simulink model "reduce_emf_user_cleanup"  (R2024b)
settings: Solver=FixedStepAuto  StartTime=0.0  StopTime=10  FixedStep=Tsim  RelTol=1e-4  EnableMultiTasking=on
InitFcn:
  | clc;
  | clear;
  | %% Parameters of the motor
  | Tsim = 1e-6;
  | Tpwm=1e-4;
  | Ts = 1e-4;
  | R = 1.8665;
  | Rs=1.8665;
  | Ls=8.96e-3;
  | Ld = 8.96e-3;
  | Lq = 8.96e-3;
  | L1=(Ld +Lq )/2;
  | L2=(Lq -Ld )/2;
  | flux = 0.21;
  | F=0.00008;
  | J=0.003;
  | Np=4;
  | fpwm = 10e3;
  | Vdc=311;
  | wn=100;
  | %% Controller limiter                                                           % Maximum torque (Nm)
  | I_max = 7.5;                                                    % Maximum current (A)
  | V_max = Vdc/sqrt(3);
  | 
  | 
  | %% 转速环电流环带宽
  | wspd=20;
  | wcur=500;
  | 
  | %% LESO
  | w0=10000;
  | beta1=2*w0-R/Ld;
  | beta2=w0*w0;
  | %% IF启动
  | Iq_if=7;
  | we_if_acc=300;
  | we_if_max=180;
  | we_switch=150;
model workspace (MAT data in the model file):
  new = 0
undefined symbols (not defined in the file or in its folder): DiscIntNeverNeededParam, dspblkCoreblockFVToolHelper, gcbh
libraries: spsDCVoltageSourceLib x1, spsGroundLib x1, spsPermanentMagnetSynchronousMachineLib x1, spsUniversalBridgeLib x1, spspowerguiLib x1, simulink x1
(part 1 of 2)
settings Model: SimulationMode=accelerator  Creator=Lenovo  LastModifiedBy=azx
settings SolverCC: AlgebraicLoopSolver=TrustRegion
settings DataIOCC: ReturnWorkspaceOutputs=off
settings OptimizationCC: ReuseModelBlockBuffer=off
settings DebuggingCC: UnconnectedInputMsg=warning  UnconnectedOutputMsg=warning  UnconnectedLineMsg=warning
settings ModelReferenceCC: EnableRefExpFcnMdlSchedulingChecks=on
settings RTWCC: GPUComputeCapability=3.5

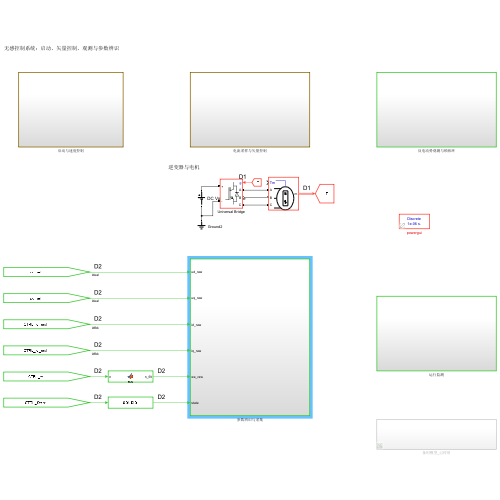
[thumbnail: Simulink's stored preview of the top-level diagram]
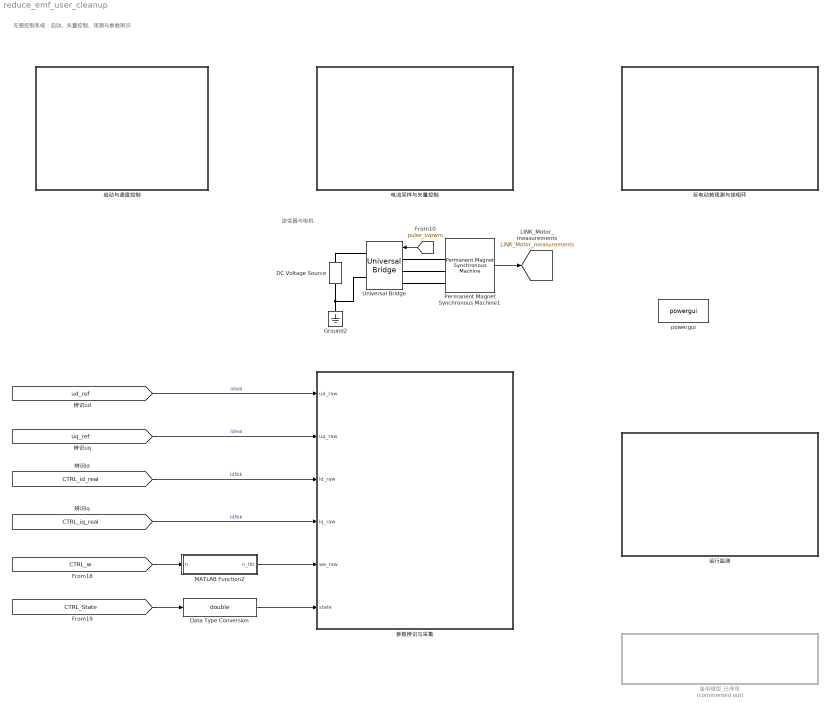
== system reduce_emf_user_cleanup ==
  note: 无感控制系统：启动、矢量控制、观测与参数辨识
  note: 逆变器与电机
  DC Voltage Source : spsDCVoltageSourceLib/DC Voltage Source  Amplitude=Vdc  Measurements=None
  Data Type Conversion : DataTypeConversion  OutDataTypeStr=double  SaturateOnIntegerOverflow=off  RndMeth=Floor
  Ground2 : spsGroundLib/Ground  LConnTagsString=a
  MATLAB Function2 : MATLAB Function  TreatAsAtomicUnit=on
  Permanent Magnet Synchronous Machine1 : spsPermanentMagnetSynchronousMachineLib/Permanent Magnet Synchronous Machine  NbPhases=3  FluxDistribution=Sinusoidal  RotorType=Salient-pole  MechanicalLoad=Torque Tm  PresetModel=No  ShowDetailedParameters=on  MeasurementBus=off  Resistance=R  Inductance=8.5e-3  dqInductances=[Ld,Lq]  La=Ld  MachineConstant=Flux linkage established by magnets (V.s)  Flux=0.21  VoltageCst=152.3591  TorqueCst=1.26  Flat=120  Mechanical=[0.03 2e-2 Np 0]  PolePairs=4  InitialConditions=[0,0, 0,0]  InitialConditions5ph=[0 0 0 0 0 0]  RefAngle=Aligned with phase A axis (original Park)  IterativeDiscreteModel=Trapezoidal non iterative  TsBlock=-1  TsPowergui=0
  Universal Bridge : spsUniversalBridgeLib/Universal Bridge  Arms=3  SnubberResistance=1e5  SnubberCapacitance=inf  Device=IGBT / Diodes  Ron=1e-3  Lon=0  ForwardVoltages="[  0  0  ]"  ForwardVoltage=0  GTOparameters=[ 10e-6 , 20e-6 ]  IGBTparameters=[ 1e-6 , 2e-6 ]  Measurements=None  Measurements_2=None  converterType=Rectifier
  powergui : spspowerguiLib/powergui  Priority=1  SimulationMode=Discrete  SampleTime=Tsim  frequency=60  Iterations=50  frequencyindice=0  Pbase=100e6  ErrMax=1e-4  UnitsV=kV  UnitsW=MW  buscounter=0  FunctionMessages=off  echomessages=off  EnableUseOfTLC=off  CurrentSourceSwitches=off  DisableSnubberDevices=off  DisableRonSwitches=off  DisableVfSwitches=off  DisplayEquations=off  AutomaticDiscreteSolvers=off  SolverType=Tustin/Backward Euler (TBE)  Interpol=off  ExternalGateDelay=off  methode=off  Ts=100  x0status=blocks  SPID=on  SwTol=0  HookPort=off  NonlinearTolerance=1e-4  nMaxIteration=100  ContinueOnMaxIteration=off  RestoreLinks=warning  ResistiveCurrentMeasurement=off  Frange=[0:2:500]  Ylog=off  Xlog=on  ShowGrid=off  save=off  variable=ZData  structure=0  ZoomFFT=off  StartTime=0.0  cycles=1  DisplayStyle=1  fundamental=60  FreqAxis=off  MaxFrequency=1000  frequencyindicesteady=1  RmsSteady=1  display=off
  参数辨识与采集 : Subsystem
  反电动势观测与锁相环 : Subsystem  Description=仅整理原计算块与信号标签；虚拟子系统，不增加采样、延迟或执行条件。
  启动与速度控制 : Subsystem  Description=仅整理原计算块与信号标签；虚拟子系统，不增加采样、延迟或执行条件。
  备用模型_已停用 : Subsystem  Commented=on
  电流采样与矢量控制 : Subsystem  Description=仅整理原计算块与信号标签；虚拟子系统，不增加采样、延迟或执行条件。
  运行监测 : Subsystem  Description=仅整理原计算块与信号标签；虚拟子系统，不增加采样、延迟或执行条件。
  tag scope: LINK_Motor_measurements=global
  wires:
  [pulse_svpwm] -> Universal Bridge/1
  Permanent Magnet Synchronous Machine1/1 -> [LINK_Motor_measurements]
  [CTRL_w] -> MATLAB Function2/1(n)
  [CTRL_State] -> Data Type Conversion/1
  [ud_ref] -> 参数辨识与采集/1(ud_raw)  "ideal"
  [uq_ref] -> 参数辨识与采集/2(uq_raw)  "ideal"
  [CTRL_id_real] -> 参数辨识与采集/3(id_raw)  "idfbk"
  [CTRL_iq_real] -> 参数辨识与采集/4(iq_raw)  "idfbk"
  MATLAB Function2/1(n_filt) -> 参数辨识与采集/5(we_raw)
  Data Type Conversion/1 -> 参数辨识与采集/6(state)
  connections:
  DC Voltage Source/RConn1 -- Universal Bridge/RConn1
  Permanent Magnet Synchronous Machine1/LConn1 -- Universal Bridge/LConn1
  Permanent Magnet Synchronous Machine1/LConn2 -- Universal Bridge/LConn2
  Permanent Magnet Synchronous Machine1/LConn3 -- Universal Bridge/LConn3
  Universal Bridge/RConn2 -- DC Voltage Source/LConn1 -- Ground2/LConn1

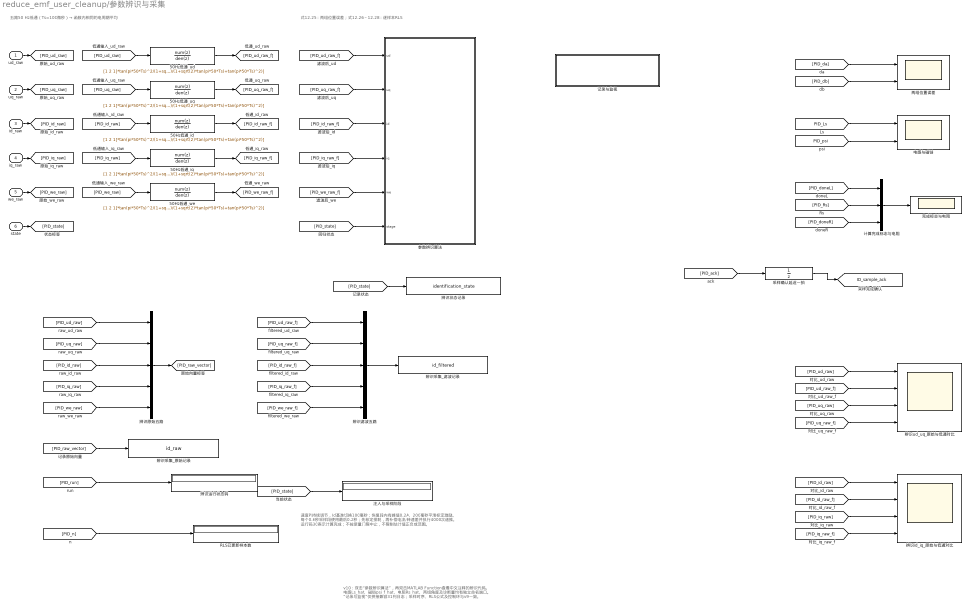
== system reduce_emf_user_cleanup/参数辨识与采集 ==
  note: 五路50 Hz低通（Ts=100微秒）→ 函数内相同的电周期平均
  note: 式12.25：两组位置误差；式12.26～12.28：逐样本RLS
  note: 速度PI持续调节，Id基准切换100毫秒；恢复段内有峰值0.2A、200毫秒平滑标定激励。
      | 每个0.6秒采样段使用最后0.2秒；先标定损耗，再补偿电流/转速差并执行4000次递推。
      | 运行码30表示计算完成；不按质量门限中止，不限制估计值正负或范围。
  note: v10：双击“参数辨识算法”，再双击MATLAB Function查看中文注释的辨识代码。
      | 电感Ls_hat、磁链psi_f_hat、电阻Rs_hat、两组角度及诊断量均有独立命名端口。
      | “记录与监视”仅拼接兼容31列日志；采样时序、RLS公式及控制环与v9一致。
  ud_raw : Inport
  uq_raw : Inport  Port=2
  id_raw : Inport  Port=3
  iq_raw : Inport  Port=4
  we_raw : Inport  Port=5
  state : Inport  Port=6
  50Hz低通_id : DiscreteTransferFcn  Description=输入已是Ts=100us；同速率二阶Butterworth低通，不作升采样，不声称恢复上游已混叠信息。  Numerator=[1 2 1]*tan(pi*50*Ts)^2/(1+sqrt(2)*tan(pi*50*Ts)+tan(pi*50*Ts)^2)  Denominator=[1 2*(tan(pi*50*Ts)^2-1)/(1+sqrt(2)*tan(pi*50*Ts)+tan(pi*50*Ts)^2) (1-sqrt(2)*tan(pi*50*Ts)+tan(pi*50*Ts)^2)/(1+sqrt(2)*tan(pi*50*Ts)+tan(pi*50*Ts)^2)]  SampleTime=Ts
  50Hz低通_iq : DiscreteTransferFcn  Description=输入已是Ts=100us；同速率二阶Butterworth低通，不作升采样，不声称恢复上游已混叠信息。  Numerator=[1 2 1]*tan(pi*50*Ts)^2/(1+sqrt(2)*tan(pi*50*Ts)+tan(pi*50*Ts)^2)  Denominator=[1 2*(tan(pi*50*Ts)^2-1)/(1+sqrt(2)*tan(pi*50*Ts)+tan(pi*50*Ts)^2) (1-sqrt(2)*tan(pi*50*Ts)+tan(pi*50*Ts)^2)/(1+sqrt(2)*tan(pi*50*Ts)+tan(pi*50*Ts)^2)]  SampleTime=Ts
  50Hz低通_ud : DiscreteTransferFcn  Description=输入已是Ts=100us；同速率二阶Butterworth低通，不作升采样，不声称恢复上游已混叠信息。  LoadFcn=dspblkCoreblockFVToolHelper(gcbh,'load');  Numerator=[1 2 1]*tan(pi*50*Ts)^2/(1+sqrt(2)*tan(pi*50*Ts)+tan(pi*50*Ts)^2)  Denominator=[1 2*(tan(pi*50*Ts)^2-1)/(1+sqrt(2)*tan(pi*50*Ts)+tan(pi*50*Ts)^2) (1-sqrt(2)*tan(pi*50*Ts)+tan(pi*50*Ts)^2)/(1+sqrt(2)*tan(pi*50*Ts)+tan(pi*50*Ts)^2)]  SampleTime=Ts
      settings: CopyFcn=dspblkCoreblockFVToolHelper(gcbh,'copy');  DeleteFcn=dspblkCoreblockFVToolHelper(gcbh,'close');  ModelCloseFcn=dspblkCoreblockFVToolHelper(gcbh,'close');  PreSaveFcn=dspblkCoreblockFVToolHelper(gcbh,'presave');  PostSaveFcn=dspblkCoreblockFVToolHelper(gcbh,'postsave');  CloseFcn=dspblkCoreblockFVToolHelper(gcbh,'close');
  50Hz低通_uq : DiscreteTransferFcn  Description=输入已是Ts=100us；同速率二阶Butterworth低通，不作升采样，不声称恢复上游已混叠信息。  Numerator=[1 2 1]*tan(pi*50*Ts)^2/(1+sqrt(2)*tan(pi*50*Ts)+tan(pi*50*Ts)^2)  Denominator=[1 2*(tan(pi*50*Ts)^2-1)/(1+sqrt(2)*tan(pi*50*Ts)+tan(pi*50*Ts)^2) (1-sqrt(2)*tan(pi*50*Ts)+tan(pi*50*Ts)^2)/(1+sqrt(2)*tan(pi*50*Ts)+tan(pi*50*Ts)^2)]  SampleTime=Ts
  50Hz低通_we : DiscreteTransferFcn  Description=输入已是Ts=100us；同速率二阶Butterworth低通，不作升采样，不声称恢复上游已混叠信息。  Numerator=[1 2 1]*tan(pi*50*Ts)^2/(1+sqrt(2)*tan(pi*50*Ts)+tan(pi*50*Ts)^2)  Denominator=[1 2*(tan(pi*50*Ts)^2-1)/(1+sqrt(2)*tan(pi*50*Ts)+tan(pi*50*Ts)^2) (1-sqrt(2)*tan(pi*50*Ts)+tan(pi*50*Ts)^2)/(1+sqrt(2)*tan(pi*50*Ts)+tan(pi*50*Ts)^2)]  SampleTime=Ts
  RLS已更新样本数 : Display
  两组位置误差 : Scope  NumInputPorts=2
  参数辨识算法 : Subsystem
  完成标志与电阻 : Scope
  注入与采样阶段 : Display
  电感与磁链 : Scope  NumInputPorts=2
  计算完成标志与电阻 : Mux  Inputs=3
  记录与监视 : Subsystem  Description=记录顺序：[Ls psi Rs da db doneL doneR run n ack R0 V0]。
  辨识id_iq_原始与低通对比 : Scope
  辨识ud_uq_原始与低通对比 : Scope
  辨识原始五路 : Mux  Inputs=5
  辨识滤波五路 : Mux  Inputs=5
  辨识状态记录 : ToWorkspace  VariableName=identification_state  SaveFormat=Structure With Time  SampleTime=Ts
  辨识运行状态码 : Display
  辨识采集_原始记录 : ToWorkspace  VariableName=id_raw  SaveFormat=Structure With Time  SampleTime=Ts
  辨识采集_滤波记录 : ToWorkspace  VariableName=id_filtered  SaveFormat=Structure With Time  SampleTime=Ts
  采样确认延迟一拍 : UnitDelay  SampleTime=Ts
  tag scope: ID_sample_ack=global
  wires:
  [PID_state] -> 辨识状态记录/1
  [PID_da] -> 两组位置误差/1
  [PID_db] -> 两组位置误差/2
  [PID_Ls] -> 电感与磁链/1
  [PID_psi] -> 电感与磁链/2
  [PID_doneL] -> 计算完成标志与电阻/1
  [PID_Rs] -> 计算完成标志与电阻/2
  [PID_doneR] -> 计算完成标志与电阻/3
  计算完成标志与电阻/1 -> 完成标志与电阻/1
  [PID_ud_raw] -> 辨识原始五路/1
  [PID_uq_raw] -> 辨识原始五路/2
  [PID_id_raw] -> 辨识原始五路/3
  [PID_iq_raw] -> 辨识原始五路/4
  [PID_we_raw] -> 辨识原始五路/5
  辨识滤波五路/1 -> 辨识采集_滤波记录/1
  [PID_ud_raw_f] -> 辨识滤波五路/1
  [PID_uq_raw_f] -> 辨识滤波五路/2
  [PID_id_raw_f] -> 辨识滤波五路/3
  [PID_iq_raw_f] -> 辨识滤波五路/4
  [PID_we_raw_f] -> 辨识滤波五路/5
  [PID_ud_raw] -> 辨识ud_uq_原始与低通对比/1
  [PID_ud_raw_f] -> 辨识ud_uq_原始与低通对比/2
  [PID_uq_raw] -> 辨识ud_uq_原始与低通对比/3
  [PID_uq_raw_f] -> 辨识ud_uq_原始与低通对比/4
  [PID_id_raw] -> 辨识id_iq_原始与低通对比/1
  [PID_id_raw_f] -> 辨识id_iq_原始与低通对比/2
  [PID_iq_raw] -> 辨识id_iq_原始与低通对比/3
  [PID_iq_raw_f] -> 辨识id_iq_原始与低通对比/4
  辨识原始五路/1 -> [PID_raw_vector]
  [PID_raw_vector] -> 辨识采集_原始记录/1
  采样确认延迟一拍/1 -> [ID_sample_ack]
  [PID_state] -> 注入与采样阶段/1
  ud_raw/1 -> [PID_ud_raw]
  [PID_ud_raw] -> 50Hz低通_ud/1
  50Hz低通_ud/1 -> [PID_ud_raw_f]
  uq_raw/1 -> [PID_uq_raw]
  [PID_uq_raw] -> 50Hz低通_uq/1
  50Hz低通_uq/1 -> [PID_uq_raw_f]
  id_raw/1 -> [PID_id_raw]
  [PID_id_raw] -> 50Hz低通_id/1
  50Hz低通_id/1 -> [PID_id_raw_f]
  iq_raw/1 -> [PID_iq_raw]
  [PID_iq_raw] -> 50Hz低通_iq/1
  50Hz低通_iq/1 -> [PID_iq_raw_f]
  we_raw/1 -> [PID_we_raw]
  [PID_we_raw] -> 50Hz低通_we/1
  50Hz低通_we/1 -> [PID_we_raw_f]
  state/1 -> [PID_state]
  [PID_ud_raw_f] -> 参数辨识算法/1(ud)
  [PID_uq_raw_f] -> 参数辨识算法/2(uq)
  [PID_id_raw_f] -> 参数辨识算法/3(id)
  [PID_iq_raw_f] -> 参数辨识算法/4(iq)
  [PID_we_raw_f] -> 参数辨识算法/5(we)
  [PID_state] -> 参数辨识算法/6(stage)
  [PID_ack] -> 采样确认延迟一拍/1
  [PID_run] -> 辨识运行状态码/1
  [PID_n] -> RLS已更新样本数/1

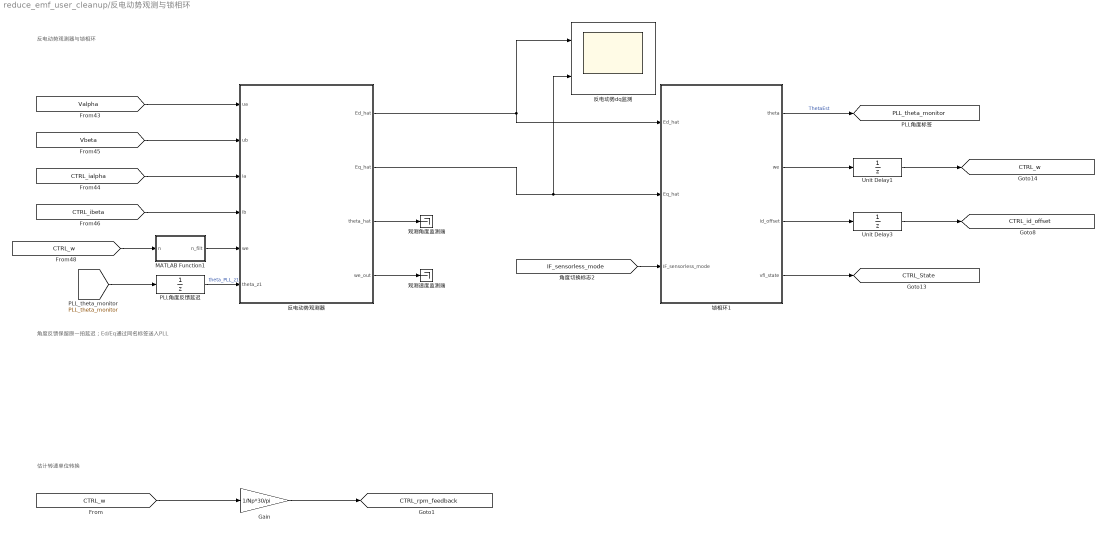
== system reduce_emf_user_cleanup/反电动势观测与锁相环 ==
  note: 反电动势观测器与锁相环
  note: 角度反馈保留原一拍延迟；Ed/Eq通过同名标签送入PLL
  note: 估计转速单位转换
  Gain : Gain  Gain=1/Np*30/pi
  MATLAB Function1 : MATLAB Function  Description=旁路100Hz低通，使用原有一拍延迟PLL速度，与角度反馈推进严格同拍。  TreatAsAtomicUnit=on
  PLL角度反馈延迟 : UnitDelay  SampleTime=1e-4
  Unit Delay1 : UnitDelay  SampleTime=-1  HasFrameUpgradeWarning=on
  Unit Delay3 : UnitDelay  SampleTime=-1  HasFrameUpgradeWarning=on
  反电动势dq监测 : Scope  NumInputPorts=2
  反电动势观测器 : MATLAB Function  Description=按文档式12.5-12.7、图12.2实现dq降阶反电动势观测器，Ed/Eq直接送PLL。  TreatAsAtomicUnit=on
  观测角度监测端 : Terminator
  观测速度监测端 : Terminator
  锁相环1 : Subsystem  Description=v9：速度PI不冻结；采样段0.6秒，Id恢复段1秒含0.2A平滑标定激励，正式采样前恢复650毫秒。
  tag scope: CTRL_State=global, CTRL_id_offset=global, CTRL_rpm_feedback=global, CTRL_w=global, PLL_theta_monitor=global
  wires:
  Gain/1 -> [CTRL_rpm_feedback]
  Unit Delay1/1 -> [CTRL_w]
  锁相环1/1(theta) -> [PLL_theta_monitor]  "ThetaEst"
  Unit Delay3/1 -> [CTRL_id_offset]
  锁相环1/4(vfl_state) -> [CTRL_State]
  [Valpha] -> 反电动势观测器/1(ua)
  反电动势观测器/2(Eq_hat) -> 反电动势dq监测/2, 锁相环1/2(Eq_hat)
  [Vbeta] -> 反电动势观测器/2(ub)
  [CTRL_ialpha] -> 反电动势观测器/3(ia)
  [CTRL_ibeta] -> 反电动势观测器/4(ib)
  反电动势观测器/1(Ed_hat) -> 锁相环1/1(Ed_hat), 反电动势dq监测/1
  锁相环1/2(we) -> Unit Delay1/1
  [CTRL_w] -> MATLAB Function1/1(n)
  [CTRL_w] -> Gain/1
  [PLL_theta_monitor] -> PLL角度反馈延迟/1
  [IF_sensorless_mode] -> 锁相环1/3(IF_sensorless_mode)
  锁相环1/3(id_offset) -> Unit Delay3/1
  MATLAB Function1/1(n_filt) -> 反电动势观测器/5("we ")
  PLL角度反馈延迟/1 -> 反电动势观测器/6(theta_z1)  "theta_PLL_z1"
  反电动势观测器/3(theta_hat) -> 观测角度监测端/1
  反电动势观测器/4(we_out) -> 观测速度监测端/1

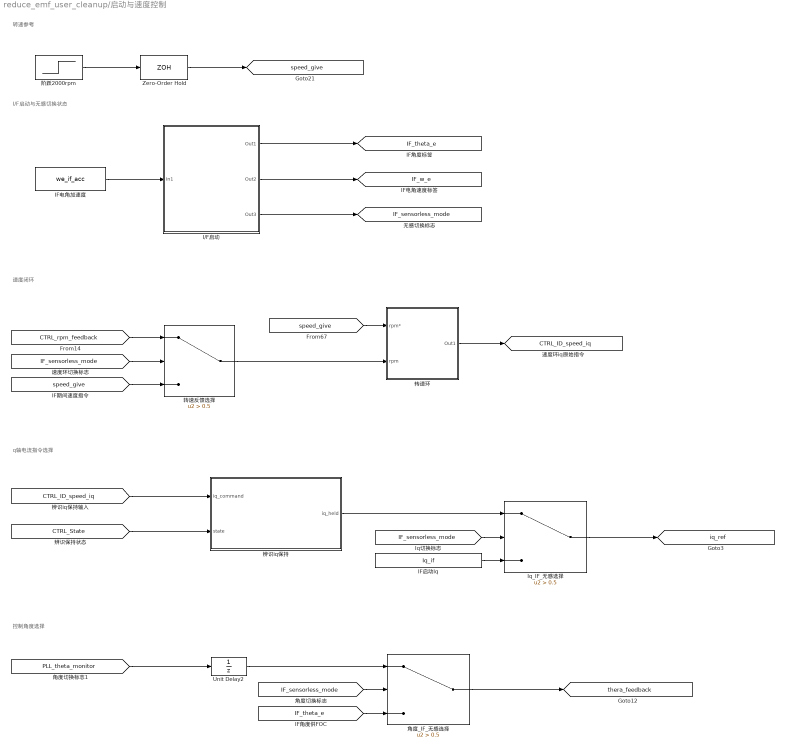
== system reduce_emf_user_cleanup/启动与速度控制 ==
  note: 转速参考
  note: I/F启动与无感切换状态
  note: 速度闭环
  note: q轴电流指令选择
  note: 控制角度选择
  I/F启动 : Subsystem
  IF启动Iq : Constant  Value=Iq_if  SampleTime=Ts
  IF电角加速度 : Constant  Value=we_if_acc  SampleTime=Ts
  Iq_IF_无感选择 : Switch  Criteria=u2 > Threshold  Threshold=0.5
  Unit Delay2 : UnitDelay  SampleTime=-1  HasFrameUpgradeWarning=on
  Zero-Order Hold : ZeroOrderHold  SampleTime=1e-4
  角度_IF_无感选择 : Switch  Criteria=u2 > Threshold  Threshold=0.5
  转速反馈选择 : Switch  Criteria=u2 > Threshold  Threshold=0.5
  转速环 : Subsystem
  辨识iq保持 : Subsystem
  阶跃2000rpm : Step  Time=2  Before=500  After=500  SampleTime=0
  tag scope: CTRL_ID_speed_iq=global, IF_sensorless_mode=global, IF_theta_e=global, IF_w_e=global, iq_ref=global, speed_give=global, thera_feedback=global
  wires:
  Zero-Order Hold/1 -> [speed_give]
  角度_IF_无感选择/1 -> [thera_feedback]
  Iq_IF_无感选择/1 -> [iq_ref]
  I/F启动/1(Out1) -> [IF_theta_e]
  I/F启动/2(Out2) -> [IF_w_e]
  I/F启动/3(Out3) -> [IF_sensorless_mode]
  转速环/1(Out1) -> [CTRL_ID_speed_iq]
  阶跃2000rpm/1 -> Zero-Order Hold/1
  [speed_give] -> 转速环/1(rpm*)
  [IF_sensorless_mode] -> Iq_IF_无感选择/2
  IF启动Iq/1 -> Iq_IF_无感选择/3
  [CTRL_rpm_feedback] -> 转速反馈选择/1
  [IF_sensorless_mode] -> 转速反馈选择/2
  [speed_give] -> 转速反馈选择/3
  转速反馈选择/1 -> 转速环/2(rpm)
  [IF_sensorless_mode] -> 角度_IF_无感选择/2
  [IF_theta_e] -> 角度_IF_无感选择/3
  [PLL_theta_monitor] -> Unit Delay2/1
  IF电角加速度/1 -> I/F启动/1(In1)
  Unit Delay2/1 -> 角度_IF_无感选择/1
  [CTRL_State] -> 辨识iq保持/2(state)
  辨识iq保持/1(iq_held) -> Iq_IF_无感选择/1
  [CTRL_ID_speed_iq] -> 辨识iq保持/1(iq_command)

== system reduce_emf_user_cleanup/备用模型_已停用 ==
  Step1 : Step  Time=0.5  Before=8.5  After=8.5  SampleTime=0
  Subsystem : Subsystem  Commented=on
  备用输入1 : Ground
  备用输入2 : Ground
  备用输出1 : Terminator
  备用输出2 : Terminator
  未启用的备用负载 : Terminator
  wires:
  备用输入1/1 -> Subsystem/1(ea)
  备用输入2/1 -> Subsystem/2(eb)
  Subsystem/1(theta) -> 备用输出1/1
  Subsystem/2(we) -> 备用输出2/1
  Step1/1 -> 未启用的备用负载/1

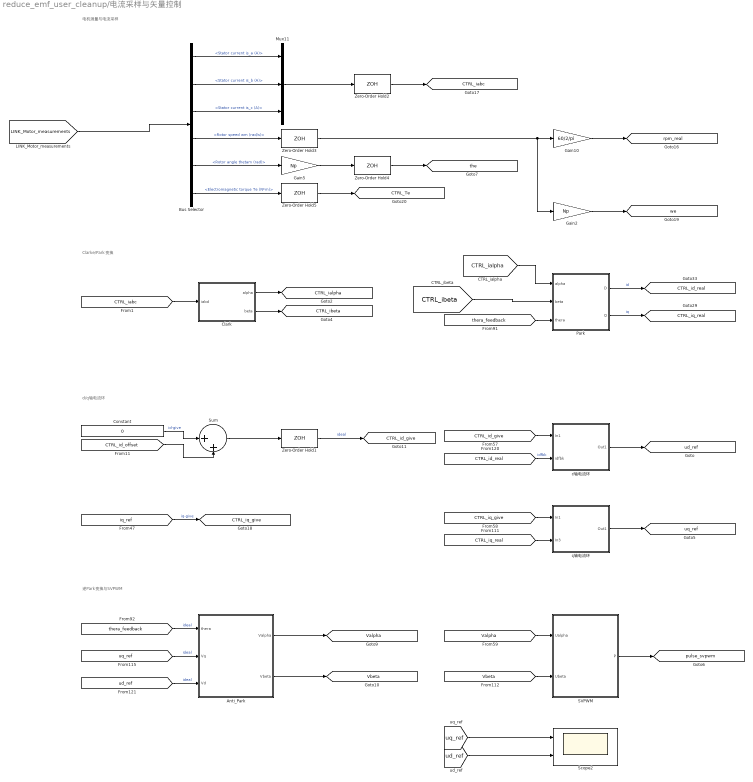
== system reduce_emf_user_cleanup/电流采样与矢量控制 ==
  note: 电机测量与电流采样
  note: Clarke/Park变换
  note: d/q轴电流环
  note: 逆Park变换与SVPWM
  Anti_Park : Subsystem
  Bus Selector : BusSelector  OutputSignals=Stator current is_a (A),Stator current is_b (A),Stator current is_c (A),Rotor speed wm (rad/s),Rotor angle thetam (rad),Electromagnetic torque Te (N*m)
  Clark : Subsystem
  Constant : Constant  Value=0
  Gain10 : Gain  Gain=60/2/pi
  Gain2 : Gain  Gain=Np
  Gain5 : Gain  Gain=Np
  Mux11 : Mux  Inputs=3
  Park : Subsystem
  SVPWM : Subsystem
  Scope2 : Scope  NumInputPorts=2
  Sum : Sum  Inputs=|++
  Zero-Order Hold{1..5} (5 alike) : ZeroOrderHold  SampleTime=1e-4
  d轴电流环 : Subsystem
  q轴电流环 : Subsystem
  tag scope: CTRL_Te=global, CTRL_iabc=global, CTRL_ialpha=global, CTRL_ibeta=global, CTRL_id_give=global, CTRL_id_real=global, CTRL_iq_give=global, CTRL_iq_real=global, Valpha=global, Vbeta=global, pulse_svpwm=global, rpm_real=global, the=global, ud_ref=global, uq_ref=global, we=global
  wires:
  Clark/2(beta) -> [CTRL_ibeta]
  Clark/1(alpha) -> [CTRL_ialpha]
  Park/1(D) -> [CTRL_id_real]  "id"
  Park/2(Q) -> [CTRL_iq_real]  "iq"
  Zero-Order Hold1/1 -> [CTRL_id_give]  "ideal"
  Zero-Order Hold5/1 -> [CTRL_Te]
  Gain2/1 -> [we]
  Zero-Order Hold2/1 -> [CTRL_iabc]
  Gain10/1 -> [rpm_real]
  Zero-Order Hold4/1 -> [the]
  Anti_Park/1(Valpha) -> [Valpha]
  Anti_Park/2(Vbeta) -> [Vbeta]
  q轴电流环/1(Out1) -> [uq_ref]
  d轴电流环/1(Out1) -> [ud_ref]
  SVPWM/1(P) -> [pulse_svpwm]
  [iq_ref] -> [CTRL_iq_give]  "iq-give"
  [CTRL_ibeta] -> Park/2(beta)
  [CTRL_ialpha] -> Park/1(alpha)
  [thera_feedback] -> Park/3(thera)
  [thera_feedback] -> Anti_Park/1(thera)  "ideal"
  [ud_ref] -> Scope2/2
  [ud_ref] -> Anti_Park/3(Vd)  "ideal"
  [uq_ref] -> Scope2/1
  [uq_ref] -> Anti_Park/2(Vq)  "ideal"
  [CTRL_iabc] -> Clark/1(iabd)
  Bus Selector/1 -> Mux11/1  "<Stator current is_a (A)>"
  Bus Selector/3 -> Mux11/3  "<Stator current is_c (A)>"
  Zero-Order Hold3/1 -> Gain2/1, Gain10/1
  Mux11/1 -> Zero-Order Hold2/1
  Bus Selector/2 -> Mux11/2  "<Stator current is_b (A)>"
  Bus Selector/5 -> Gain5/1  "<Rotor angle thetam (rad)>"
  Bus Selector/4 -> Zero-Order Hold3/1  "<Rotor speed wm (rad/s)>"
  Bus Selector/6 -> Zero-Order Hold5/1  "<Electromagnetic torque Te (N*m)>"
  [LINK_Motor_measurements] -> Bus Selector/1
  Gain5/1 -> Zero-Order Hold4/1
  [CTRL_iq_give] -> q轴电流环/1(In1)
  [CTRL_iq_real] -> q轴电流环/2(In3)
  [CTRL_id_give] -> d轴电流环/1(In1)
  [CTRL_id_real] -> d轴电流环/2(idfbk)  "idfbk"
  [Valpha] -> SVPWM/1(Ualpha)
  [Vbeta] -> SVPWM/2(Ubeta)
  Sum/1 -> Zero-Order Hold1/1
  Constant/1 -> Sum/1  "id-give"
  [CTRL_id_offset] -> Sum/2

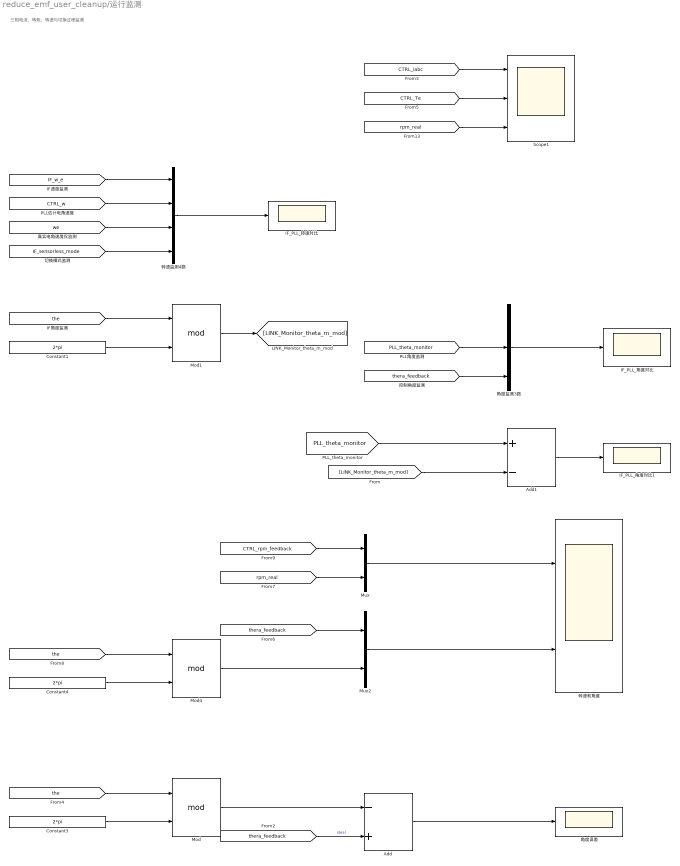
== system reduce_emf_user_cleanup/运行监测 ==
  note: 三相电流、转矩、转速与切换过程监测
  Add : Sum  Inputs=-+
  Add1 : Sum  Inputs=+-
  Constant1 : Constant  Value=2*pi
  Constant3 : Constant  Value=2*pi
  Constant4 : Constant  Value=2*pi
  IF_PLL_角度对比 : Scope
  IF_PLL_角度对比1 : Scope
  IF_PLL_转速对比 : Scope
  Mod : Math  Operator=mod
  Mod1 : Math  Operator=mod
  Mod4 : Math  Operator=mod
  Mux : Mux  Inputs=2
  Mux2 : Mux  Inputs=2
  Scope1 : Scope  NumInputPorts=3
  角度监测3路 : Mux  Inputs=3
  角度误差 : Scope
  转速和角度 : Scope  NumInputPorts=2
  转速监测4路 : Mux
  wires:
  [CTRL_rpm_feedback] -> Mux/1
  [rpm_real] -> Mux/2
  [thera_feedback] -> Mux2/1
  Mux2/1 -> 转速和角度/2
  Mux/1 -> 转速和角度/1
  [the] -> Mod/1
  Constant3/1 -> Mod/2
  Mod/1 -> Add/1
  Add/1 -> 角度误差/1
  [thera_feedback] -> Add/2  "ideal"
  [the] -> Mod4/1
  Constant4/1 -> Mod4/2
  Mod4/1 -> Mux2/2
  [rpm_real] -> Scope1/3
  [CTRL_Te] -> Scope1/2
  [CTRL_iabc] -> Scope1/1
  [IF_w_e] -> 转速监测4路/1
  [CTRL_w] -> 转速监测4路/2
  [we] -> 转速监测4路/3
  [IF_sensorless_mode] -> 转速监测4路/4
  转速监测4路/1 -> IF_PLL_转速对比/1
  [PLL_theta_monitor] -> Add1/1
  [PLL_theta_monitor] -> 角度监测3路/2
  [thera_feedback] -> 角度监测3路/3
  角度监测3路/1 -> IF_PLL_角度对比/1
  Add1/1 -> IF_PLL_角度对比1/1
  [the] -> Mod1/1
  Constant1/1 -> Mod1/2
  Mod1/1 -> [LINK_Monitor_theta_m_mod]
  [LINK_Monitor_theta_m_mod] -> Add1/2

== system reduce_emf_user_cleanup/参数辨识与采集/参数辨识算法 ==
  ud : Inport
  uq : Inport  Port=2
  id : Inport  Port=3
  iq : Inport  Port=4
  we : Inport  Port=5
  stage : Inport  Port=6
  Scope : Scope  NumInputPorts=2
  参数辨识 : MATLAB Function  Description=采样存储→正负注入求角度→逐样本RLS→电阻计算；中文注释，12路独立短名称输出。  TreatAsAtomicUnit=on
  tag scope: PID_Ls=global, PID_psi=global
  wires:
  ud/1 -> 参数辨识/1(ud)  "ud"
  uq/1 -> 参数辨识/2(uq)  "uq"
  id/1 -> 参数辨识/3(id)  "id"
  iq/1 -> 参数辨识/4(iq)  "iq"
  we/1 -> 参数辨识/5(we)  "we"
  stage/1 -> 参数辨识/6(stage)  "stage"
  参数辨识/1(dtheta) -> [PID_Ls]  "Ls"
  参数辨识/2(dtheta1) -> [PID_psi]  "psi"
  参数辨识/3(Ls_hat) -> Scope/1
  参数辨识/4(psi_hat) -> Scope/2

== system reduce_emf_user_cleanup/参数辨识与采集/记录与监视 ==
  参数辨识结果记录 : ToWorkspace  VariableName=param_identification  SaveFormat=Structure With Time  SampleTime=Ts
  结果记录_12列 : Mux  Inputs=12
  wires:
  [PID_Ls] -> 结果记录_12列/1
  [PID_psi] -> 结果记录_12列/2
  [PID_Rs] -> 结果记录_12列/3
  [PID_da] -> 结果记录_12列/4
  [PID_db] -> 结果记录_12列/5
  [PID_doneL] -> 结果记录_12列/6
  [PID_doneR] -> 结果记录_12列/7
  [PID_run] -> 结果记录_12列/8
  [PID_n] -> 结果记录_12列/9
  [PID_ack] -> 结果记录_12列/10
  [PID_R0] -> 结果记录_12列/11
  [PID_V0] -> 结果记录_12列/12
  结果记录_12列/1 -> 参数辨识结果记录/1

== system reduce_emf_user_cleanup/反电动势观测与锁相环/锁相环1 ==
  Ed_hat : Inport
  Eq_hat : Inport  Port=2
  IF_sensorless_mode : Inport  Port=3
  MATLAB Function : MATLAB Function  TreatAsAtomicUnit=on
  theta : Outport
  we : Outport  Port=2
  id_offset : Outport  Port=3
  vfl_state : Outport  Port=4
  wires:
  Ed_hat/1 -> MATLAB Function/1(Ed_hat)
  Eq_hat/1 -> MATLAB Function/2(Eq_hat)
  MATLAB Function/1(theta) -> theta/1
  MATLAB Function/2(we) -> we/1
  IF_sensorless_mode/1 -> MATLAB Function/3(IF_sensorless_mode)
  MATLAB Function/3(id_offset) -> id_offset/1
  MATLAB Function/4(vfl_state) -> vfl_state/1
  [ID_sample_ack] -> MATLAB Function/4(sample_ack)

== system reduce_emf_user_cleanup/启动与速度控制/I//F启动 ==
  In1 : Inport
  2π : Constant  Value=2*pi  SampleTime=Ts
  Data Type Conversion : DataTypeConversion  OutDataTypeStr=double  SaturateOnIntegerOverflow=off  RndMeth=Floor
  IF角度取模 : Math  Operator=mod
  IF角度积分 : DiscreteIntegrator  SampleTime=Ts  ICPrevOutput=DiscIntNeverNeededParam  ICPrevScaledInput=DiscIntNeverNeededParam
  IF转速达到阈值 : RelationalOperator
  IF速度上限 : Saturate  UpperLimit=we_if_max  LowerLimit=0
  IF速度积分 : DiscreteIntegrator  SampleTime=Ts  ICPrevOutput=DiscIntNeverNeededParam  ICPrevScaledInput=DiscIntNeverNeededParam
  切换电角速度 : Constant  Value=we_switch  SampleTime=Ts
  Out1 : Outport
  Out2 : Outport  Port=2
  Out3 : Outport  Port=3
  wires:
  切换电角速度/1 -> IF转速达到阈值/2
  IF速度积分/1 -> IF速度上限/1
  2π/1 -> IF角度取模/2
  IF速度上限/1 -> Out2/1, IF转速达到阈值/1, IF角度积分/1
  IF角度积分/1 -> IF角度取模/1
  IF转速达到阈值/1 -> Data Type Conversion/1
  In1/1 -> IF速度积分/1
  Data Type Conversion/1 -> Out3/1
  IF角度取模/1 -> Out1/1

== system reduce_emf_user_cleanup/启动与速度控制/转速环 ==
  rpm* : Inport
  rpm : Inport  Port=2
  30speed : Subsystem  DialogController=POWERSYS.PowerSysDialog  mask(Discrete PI Controller){Kp=0.5, Ki=5, Par_Limits=[I_max -I_max], Init=0, Ts=Ts}
      mask prompts: Kp "Proportional gain (Kp):"; Ki "Integral gain (Ki):"; Par_Limits "Output limits: [ Upper   Lower ]"; Init "Output initial value:"; Ts "Sample time:"
      mask help: This block implements a discrete PI controller.
      mask init:
      | UpperLimit=Par_Limits(1);
      | LowerLimit=Par_Limits(2);
      | power_initmask();
      mask Help: This block is part of a subset of blocks in the Extras library that does not have documentation associated with it, other than the block mask description.
      mask Display: disp('PI');
  Gain : Gain  Gain=2*pi/60
  Sum : Sum  Inputs=|+-
  辨识期间暂停速度PI误差 : Switch  Criteria=u2 > Threshold  Threshold=0.5
  辨识期间零速度误差 : Constant  Value=0  SampleTime=Ts
  Out1 : Outport
  wires:
  Sum/1 -> Gain/1
  rpm*/1 -> Sum/1
  rpm/1 -> Sum/2
  Gain/1 -> 辨识期间暂停速度PI误差/3
  30speed/1(Out) -> Out1/1
  [ID_acquisition_hold] -> 辨识期间暂停速度PI误差/2
  辨识期间零速度误差/1 -> 辨识期间暂停速度PI误差/1
  辨识期间暂停速度PI误差/1 -> 30speed/1(Error)

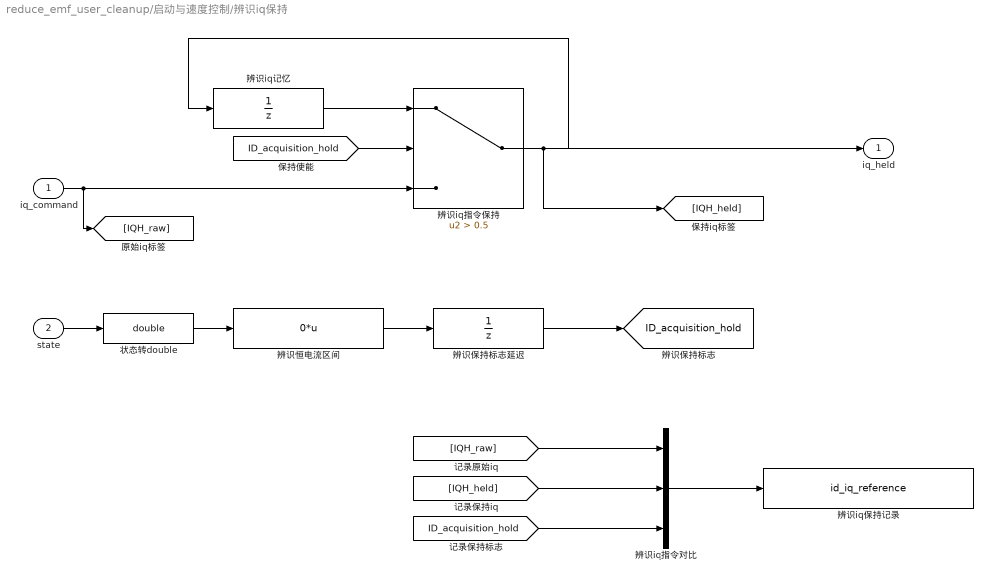
== system reduce_emf_user_cleanup/启动与速度控制/辨识iq保持 ==
  iq_command : Inport
  state : Inport  Port=2
  状态转double : DataTypeConversion  OutDataTypeStr=double
  辨识iq保持记录 : ToWorkspace  VariableName=id_iq_reference  SaveFormat=Structure With Time  SampleTime=Ts
  辨识iq指令保持 : Switch  Criteria=u2 > Threshold  Threshold=0.5
  辨识iq指令对比 : Mux  Inputs=3
  辨识iq记忆 : UnitDelay  SampleTime=Ts
  辨识保持标志延迟 : UnitDelay  SampleTime=Ts
  辨识恒电流区间 : Fcn  Description=辨识保持使能固定为0：iq直通速度PI输出，速度PI误差不再置零。  Expr=0*u
  iq_held : Outport
  tag scope: ID_acquisition_hold=global
  wires:
  state/1 -> 状态转double/1
  状态转double/1 -> 辨识恒电流区间/1
  iq_command/1 -> 辨识iq指令保持/3, [IQH_raw]
  辨识恒电流区间/1 -> 辨识保持标志延迟/1
  辨识保持标志延迟/1 -> [ID_acquisition_hold]
  [ID_acquisition_hold] -> 辨识iq指令保持/2
  辨识iq记忆/1 -> 辨识iq指令保持/1
  辨识iq指令保持/1 -> 辨识iq记忆/1, iq_held/1, [IQH_held]
  [IQH_raw] -> 辨识iq指令对比/1
  [IQH_held] -> 辨识iq指令对比/2
  [ID_acquisition_hold] -> 辨识iq指令对比/3
  辨识iq指令对比/1 -> 辨识iq保持记录/1

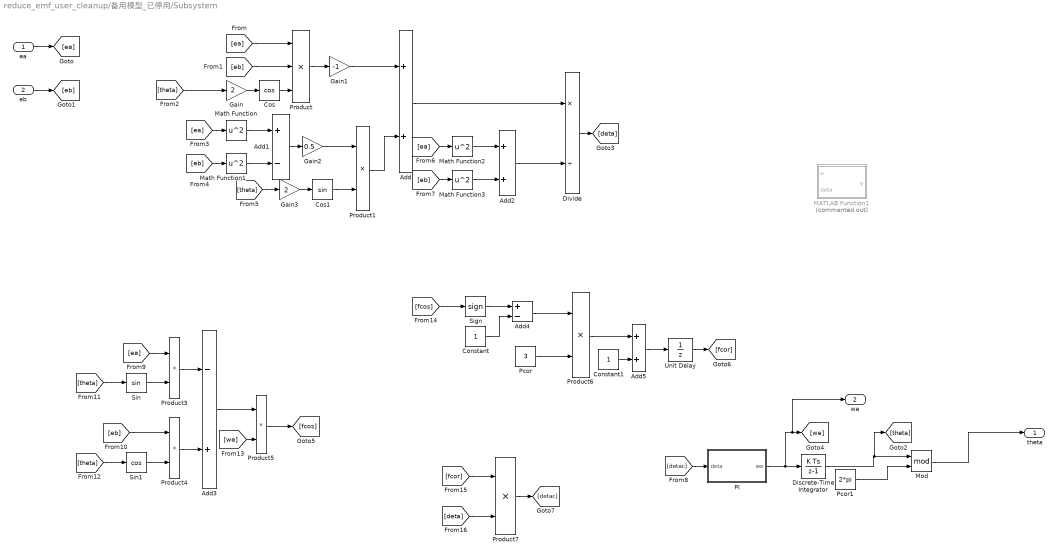
== system reduce_emf_user_cleanup/备用模型_已停用/Subsystem ==
  ea : Inport
  eb : Inport  Port=2
  Add : Sum
  Add1 : Sum  Inputs=+-
  Add2 : Sum
  Add3 : Sum  Inputs=-+
  Add4 : Sum  Inputs=+-
  Add5 : Sum
  Constant : Constant
  Constant1 : Constant
  Cos : Trigonometry  Operator=cos
  Cos1 : Trigonometry
  Discrete-Time Integrator : DiscreteIntegrator  SampleTime=-1  ICPrevOutput=DiscIntNeverNeededParam  ICPrevScaledInput=DiscIntNeverNeededParam
  Divide : Product  Inputs=*/
  Gain : Gain  Gain=2
  Gain1 : Gain  Gain=-1
  Gain2 : Gain  Gain=0.5
  Gain3 : Gain  Gain=2
  MATLAB Function1 : MATLAB Function  Commented=on  TreatAsAtomicUnit=on
  Math Function{,1..3} (4 alike) : Math  Operator=square
  Mod : Math  Operator=mod
  PI : Subsystem
  Pcor : Constant  Value=3
  Pcor1 : Constant  Value=2*pi
  Product : Product  Inputs=3
  Product{1,3..7} (6 alike) : Product
  Sign : Signum
  Sin : Trigonometry
  Sin1 : Trigonometry  Operator=cos
  Unit Delay : UnitDelay  SampleTime=-1  HasFrameUpgradeWarning=on
  theta : Outport
  we : Outport  Port=2
  wires:
  ea/1 -> [ea]
  eb/1 -> [eb]
  [ea] -> Product/1
  [eb] -> Product/2
  Cos/1 -> Product/3
  Gain/1 -> Cos/1
  [theta] -> Gain/1
  Product/1 -> Gain1/1
  Gain1/1 -> Add/1
  [ea] -> Math Function/1
  [eb] -> Math Function1/1
  Math Function/1 -> Add1/1
  Math Function1/1 -> Add1/2
  Add1/1 -> Gain2/1
  Gain2/1 -> Product1/1
  Product1/1 -> Add/2
  Cos1/1 -> Product1/2
  Gain3/1 -> Cos1/1
  [theta] -> Gain3/1
  Add/1 -> Divide/1
  Math Function3/1 -> Add2/2
  [ea] -> Math Function2/1
  [eb] -> Math Function3/1
  Math Function2/1 -> Add2/1
  [ea] -> Product3/1
  Sin/1 -> Product3/2
  [theta] -> Sin/1
  [eb] -> Product4/1
  [theta] -> Sin1/1
  Sin1/1 -> Product4/2
  Product3/1 -> Add3/1
  Product4/1 -> Add3/2
  Add3/1 -> Product5/1
  [we] -> Product5/2
  Product5/1 -> [fcos]
  [fcos] -> Sign/1
  Sign/1 -> Add4/1
  Constant/1 -> Add4/2
  Add4/1 -> Product6/1
  Pcor/1 -> Product6/2
  Product6/1 -> Add5/1
  Constant1/1 -> Add5/2
  Add5/1 -> Unit Delay/1
  [fcor] -> Product7/1
  [deta] -> Product7/2
  Product7/1 -> [detac]
  PI/1(we) -> Discrete-Time Integrator/1, we/1, [we]
  Discrete-Time Integrator/1 -> [theta], Mod/1
  Unit Delay/1 -> [fcor]
  Pcor1/1 -> Mod/2
  [detac] -> PI/1(deta)
  Add2/1 -> Divide/2
  Divide/1 -> [deta]
  Mod/1 -> theta/1

== system reduce_emf_user_cleanup/电流采样与矢量控制/Anti_Park ==
  thera : Inport
  Vq : Inport  Port=2
  Vd : Inport  Port=3
  Fcn : Fcn  Expr=cos(u[1])*u[2]-sin(u[1])*u[3]
  Fcn1 : Fcn  Expr=sin(u[1])*u[2]+cos(u[1])*u[3]
  Mux1 : Mux  Inputs=3
  Valpha : Outport
  Vbeta : Outport  Port=2
  wires:
  thera/1 -> Mux1/1
  Mux1/1 -> Fcn1/1, Fcn/1
  Vq/1 -> Mux1/3
  Fcn1/1 -> Vbeta/1
  Vd/1 -> Mux1/2
  Fcn/1 -> Valpha/1

== system reduce_emf_user_cleanup/电流采样与矢量控制/Clark ==
  iabd : Inport
  Fcn : Fcn  Expr=(u(1)-0.5*(u(2)+u(3)))*2/3
  Fcn1 : Fcn  Expr=sqrt(3)/2*(u(2)-u(3))*2/3
  alpha : Outport
  beta : Outport  Port=2
  tag scope: Ialpha_real=global, Ibeta_real=global
  wires:
  iabd/1 -> Fcn1/1, Fcn/1
  Fcn/1 -> [Ialpha_real], alpha/1
  Fcn1/1 -> [Ibeta_real], beta/1

== system reduce_emf_user_cleanup/电流采样与矢量控制/Park ==
  alpha : Inport
  beta : Inport  Port=2
  thera : Inport  Port=3
  Fcn : Fcn  Expr=u(1)*cos(u(3))+u(2)*sin(u(3))
  Fcn1 : Fcn  Expr=-u(1)*sin(u(3))+u(2)*cos(u(3))
  Mux1 : Mux  Inputs=3
  D : Outport
  Q : Outport  Port=2
  wires:
  beta/1 -> Mux1/2
  Mux1/1 -> Fcn1/1, Fcn/1
  thera/1 -> Mux1/3
  Fcn/1 -> D/1
  Fcn1/1 -> Q/1
  alpha/1 -> Mux1/1

== system reduce_emf_user_cleanup/电流采样与矢量控制/SVPWM ==
  Ualpha : Inport
  Ubeta : Inport  Port=2
  Rate Transition : RateTransition  Deterministic=off
  Rate Transition12 : RateTransition  Deterministic=off
  SVPWM : Subsystem
  P : Outport
  wires:
  Ualpha/1 -> Rate Transition/1
  Ubeta/1 -> Rate Transition12/1
  Rate Transition/1 -> SVPWM/1(alpha)
  Rate Transition12/1 -> SVPWM/2(beta)
  SVPWM/1(Pulse) -> P/1

== system reduce_emf_user_cleanup/电流采样与矢量控制/d轴电流环 ==
  In1 : Inport
  idfbk : Inport  Port=2
  30id : Subsystem  DialogController=POWERSYS.PowerSysDialog  mask(Discrete PI Controller){Kp=2*pi*wcur*Ld, Ki=2*pi*wcur*R, Par_Limits=[V_max -V_max], Init=0, Ts=Ts}
      mask prompts: Kp "Proportional gain (Kp):"; Ki "Integral gain (Ki):"; Par_Limits "Output limits: [ Upper   Lower ]"; Init "Output initial value:"; Ts "Sample time:"
      mask help: This block implements a discrete PI controller.
      mask init:
      | UpperLimit=Par_Limits(1);
      | LowerLimit=Par_Limits(2);
      | power_initmask();
      mask Help: This block is part of a subset of blocks in the Extras library that does not have documentation associated with it, other than the block mask description.
      mask Display: disp('PI');
  Sum1 : Sum  Inputs=|+-
  Sum7 : Sum  Inputs=|+-
  Out1 : Outport
  wires:
  30id/1(Out) -> Sum7/1  "ideal"
  Sum1/1 -> 30id/1(Error)
  Sum7/1 -> Out1/1
  idfbk/1 -> Sum1/2
  In1/1 -> Sum1/1

== system reduce_emf_user_cleanup/电流采样与矢量控制/q轴电流环 ==
  In1 : Inport
  In3 : Inport  Port=2
  30iq : Subsystem  DialogController=POWERSYS.PowerSysDialog  mask(Discrete PI Controller){Kp=2*pi*wcur*Lq, Ki=2*pi*wcur*R, Par_Limits=[V_max -V_max], Init=0, Ts=Ts}
      mask prompts: Kp "Proportional gain (Kp):"; Ki "Integral gain (Ki):"; Par_Limits "Output limits: [ Upper   Lower ]"; Init "Output initial value:"; Ts "Sample time:"
      mask help: This block implements a discrete PI controller.
      mask init:
      | UpperLimit=Par_Limits(1);
      | LowerLimit=Par_Limits(2);
      | power_initmask();
      mask Help: This block is part of a subset of blocks in the Extras library that does not have documentation associated with it, other than the block mask description.
      mask Display: disp('PI');
  Sum2 : Sum  Inputs=|+-
  Sum6 : Sum  Inputs=|++
  Out1 : Outport
  wires:
  In3/1 -> Sum2/2
  30iq/1(Out) -> Sum6/1  "ideal"
  Sum2/1 -> 30iq/1(Error)
  In1/1 -> Sum2/1
  Sum6/1 -> Out1/1

== system reduce_emf_user_cleanup/启动与速度控制/转速环/30speed ==
  note: Discrete PID Controller
  note: Pierre Giroux, Gilbert Sybille
      | Power System Simulation Laboratory
      | IREQ, Hydro-Quebc
  Error : Inport  SampleTime=Ts
  Add : Sum
  Add1 : Sum  Inputs=-+
  Discrete-Time Integrator : DiscreteIntegrator  InitialCondition=Init  SampleTime=Ts  UpperSaturationLimit=UpperLimit  LowerSaturationLimit=LowerLimit  ICPrevOutput=DiscIntNeverNeededParam  ICPrevScaledInput=DiscIntNeverNeededParam
  Kp1 : Gain  Gain=1/Kp  SaturateOnIntegerOverflow=on  SampleTime=Ts  OutDataTypeStr=Inherit: Same as input  ParamDataTypeStr=Inherit: Same as input
  Kp4 : Gain  Gain=Kp  SaturateOnIntegerOverflow=on  SampleTime=Ts  OutDataTypeStr=Inherit: Same as input  ParamDataTypeStr=Inherit: Same as input
  Kp5 : Gain  Gain=Ki  SaturateOnIntegerOverflow=on  SampleTime=Ts  OutDataTypeStr=Inherit: Same as input  ParamDataTypeStr=Inherit: Same as input
  Saturation2 : Saturate  UpperLimit=UpperLimit  LowerLimit=LowerLimit  SampleTime=Ts
  Sum6 : Sum  InputSameDT=on  SaturateOnIntegerOverflow=on  SampleTime=Ts  OutDataTypeStr=Inherit: Same as first input
  Zero-Order Hold : ZeroOrderHold  SampleTime=Ts
  Out : Outport  SampleTime=Ts  InitialOutput=0
  wires:
  Kp1/1 -> Add/2
  Add1/1 -> Kp1/1
  Add/1 -> Kp5/1
  Zero-Order Hold/1 -> Sum6/1
  Discrete-Time Integrator/1 -> Sum6/2
  Kp4/1 -> Zero-Order Hold/1
  Kp5/1 -> Discrete-Time Integrator/1
  Error/1 -> Kp4/1, Add/1
  Sum6/1 -> Saturation2/1, Add1/1
  Saturation2/1 -> Out/1, Add1/2

== system reduce_emf_user_cleanup/备用模型_已停用/Subsystem/PI ==
  deta : Inport
  Add : Sum
  Discrete-Time Integrator : DiscreteIntegrator  SampleTime=-1  ICPrevOutput=DiscIntNeverNeededParam  ICPrevScaledInput=DiscIntNeverNeededParam
  ki : Gain  Gain=wn^2
  kp : Gain  Gain=2*wn
  we : Outport
  wires:
  ki/1 -> Discrete-Time Integrator/1
  deta/1 -> kp/1, ki/1
  Discrete-Time Integrator/1 -> Add/1
  kp/1 -> Add/2
  Add/1 -> we/1

== system reduce_emf_user_cleanup/电流采样与矢量控制/SVPWM/SVPWM ==
  alpha : Inport
  beta : Inport  Port=2
  Demux : Demux  Outputs=6
  N Caculate : Subsystem
  Repeating Sequence : simulink/Sources/Repeating Sequence  rep_seq_t=[0 0.5*Tpwm Tpwm]  rep_seq_y=[0 0.5*Tpwm 0]
  Sabc Pulse : Subsystem
  Scope : Scope  NumInputPorts=6
  Scope1 : Scope
  T1 T2 Caculate : Subsystem
  Tc Caculate : Subsystem
  Ts : Constant  Value=Tpwm
  "Udc " : Constant  Value=Vdc
  XYZ Caculate : Subsystem
  Pulse : Outport  VectorParamsAs1DForOutWhenUnconnected=off
  wires:
  beta/1 -> N Caculate/1(beta), XYZ Caculate/1(beta)
  alpha/1 -> N Caculate/2(alpha), XYZ Caculate/2(alpha)
  XYZ Caculate/1(X) -> T1 T2 Caculate/1(X)
  XYZ Caculate/2(Y) -> T1 T2 Caculate/2(Y)
  XYZ Caculate/3(Z) -> T1 T2 Caculate/3(Z)
  Ts/1 -> XYZ Caculate/3("Ts "), Tc Caculate/3(Ts), T1 T2 Caculate/5("Ts ")
  T1 T2 Caculate/1(T1) -> Tc Caculate/1(T1)
  T1 T2 Caculate/2(T2) -> Tc Caculate/2(T2)
  Tc Caculate/3(Tc3) -> Sabc Pulse/3(Tc3)
  Sabc Pulse/1("Pulse ") -> Demux/1, Pulse/1
  "Udc "/1 -> XYZ Caculate/4(Udc)
  Repeating Sequence/1 -> Sabc Pulse/4(Wave)
  Demux/1 -> Scope/1
  Demux/2 -> Scope/2
  Demux/3 -> Scope/3
  Demux/4 -> Scope/4
  Demux/5 -> Scope/5
  Demux/6 -> Scope/6
  N Caculate/1(N) -> Scope1/1, Tc Caculate/4(N), T1 T2 Caculate/4(N)
  Tc Caculate/2(Tc2) -> Sabc Pulse/2(Tc2)
  Tc Caculate/1(Tc1) -> Sabc Pulse/1(Tc1)

== system reduce_emf_user_cleanup/电流采样与矢量控制/d轴电流环/30id ==
  note: Discrete PID Controller
  note: Pierre Giroux, Gilbert Sybille
      | Power System Simulation Laboratory
      | IREQ, Hydro-Quebc
  Error : Inport  SampleTime=Ts
  Add : Sum
  Add1 : Sum  Inputs=-+
  Discrete-Time Integrator : DiscreteIntegrator  InitialCondition=Init  SampleTime=Ts  LimitOutput=on  UpperSaturationLimit=UpperLimit  LowerSaturationLimit=LowerLimit  ICPrevOutput=DiscIntNeverNeededParam  ICPrevScaledInput=DiscIntNeverNeededParam
  Kp1 : Gain  Gain=1/Kp  SaturateOnIntegerOverflow=on  SampleTime=Ts  OutDataTypeStr=Inherit: Same as input  ParamDataTypeStr=Inherit: Same as input
  Kp4 : Gain  Gain=Kp  SaturateOnIntegerOverflow=on  SampleTime=Ts  OutDataTypeStr=Inherit: Same as input  ParamDataTypeStr=Inherit: Same as input
  Kp5 : Gain  Gain=Ki  SaturateOnIntegerOverflow=on  SampleTime=Ts  OutDataTypeStr=Inherit: Same as input  ParamDataTypeStr=Inherit: Same as input
  Saturation2 : Saturate  UpperLimit=UpperLimit  LowerLimit=LowerLimit  SampleTime=Ts
  Scope : Scope  NumInputPorts=2
  Sum6 : Sum  InputSameDT=on  SaturateOnIntegerOverflow=on  SampleTime=Ts  OutDataTypeStr=Inherit: Same as first input
  Zero-Order Hold : ZeroOrderHold  SampleTime=Ts
  Out : Outport  SampleTime=Ts  InitialOutput=0
  wires:
  Error/1 -> Kp4/1, Add/1
  Kp5/1 -> Discrete-Time Integrator/1
  Discrete-Time Integrator/1 -> Scope/2, Sum6/2
  Kp4/1 -> Zero-Order Hold/1
  Kp1/1 -> Add/2
  Add1/1 -> Kp1/1
  Sum6/1 -> Add1/1, Saturation2/1
  Add/1 -> Kp5/1
  Saturation2/1 -> Add1/2, Out/1
  Zero-Order Hold/1 -> Scope/1, Sum6/1

== system reduce_emf_user_cleanup/电流采样与矢量控制/q轴电流环/30iq ==
  note: Discrete PID Controller
  note: Pierre Giroux, Gilbert Sybille
      | Power System Simulation Laboratory
      | IREQ, Hydro-Quebc
  Error : Inport  SampleTime=Ts
  Add : Sum
  Add1 : Sum  Inputs=-+
  Discrete-Time Integrator : DiscreteIntegrator  InitialCondition=Init  SampleTime=Ts  LimitOutput=on  UpperSaturationLimit=UpperLimit  LowerSaturationLimit=LowerLimit  ICPrevOutput=DiscIntNeverNeededParam  ICPrevScaledInput=DiscIntNeverNeededParam
  Kp1 : Gain  Gain=1/Kp  SaturateOnIntegerOverflow=on  SampleTime=Ts  OutDataTypeStr=Inherit: Same as input  ParamDataTypeStr=Inherit: Same as input
  Kp4 : Gain  Gain=Kp  SaturateOnIntegerOverflow=on  SampleTime=Ts  OutDataTypeStr=Inherit: Same as input  ParamDataTypeStr=Inherit: Same as input
  Kp5 : Gain  Gain=Ki  SaturateOnIntegerOverflow=on  SampleTime=Ts  OutDataTypeStr=Inherit: Same as input  ParamDataTypeStr=Inherit: Same as input
  Saturation2 : Saturate  UpperLimit=UpperLimit  LowerLimit=LowerLimit  SampleTime=Ts
  Scope : Scope  NumInputPorts=2
  Sum6 : Sum  InputSameDT=on  SaturateOnIntegerOverflow=on  SampleTime=Ts  OutDataTypeStr=Inherit: Same as first input
  Zero-Order Hold : ZeroOrderHold  SampleTime=Ts
  Out : Outport  SampleTime=Ts  InitialOutput=0
  wires:
  Zero-Order Hold/1 -> Scope/1, Sum6/1
  Discrete-Time Integrator/1 -> Scope/2, Sum6/2
  Kp4/1 -> Zero-Order Hold/1
  Kp5/1 -> Discrete-Time Integrator/1
  Sum6/1 -> Add1/1, Saturation2/1
  Error/1 -> Kp4/1, Add/1
  Saturation2/1 -> Add1/2, Out/1
  Add1/1 -> Kp1/1
  Add/1 -> Kp5/1
  Kp1/1 -> Add/2

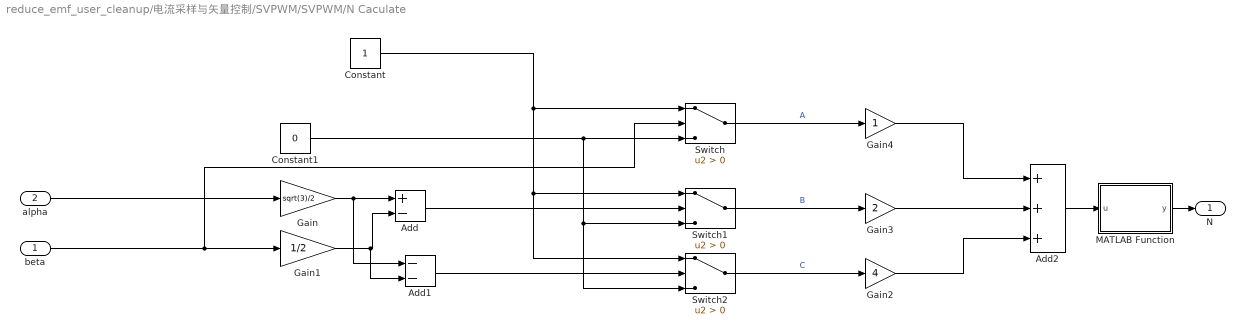
== system reduce_emf_user_cleanup/电流采样与矢量控制/SVPWM/SVPWM/N Caculate ==
  beta : Inport
  alpha : Inport  Port=2
  Add : Sum  Inputs=+-
  Add1 : Sum  Inputs=--
  Add2 : Sum  Inputs=+++
  Constant : Constant
  Constant1 : Constant  Value=0
  Gain : Gain  Gain=sqrt(3)/2
  Gain1 : Gain  Gain=1/2
  Gain2 : Gain  Gain=4
  Gain3 : Gain  Gain=2
  Gain4 : Gain
  MATLAB Function : MATLAB Function  TreatAsAtomicUnit=on
  Switch : Switch  Criteria=u2 > Threshold  SaturateOnIntegerOverflow=off  InputSameDT=off
  Switch1 : Switch  Criteria=u2 > Threshold  SaturateOnIntegerOverflow=off  InputSameDT=off
  Switch2 : Switch  Criteria=u2 > Threshold  SaturateOnIntegerOverflow=off  InputSameDT=off
  N : Outport  VectorParamsAs1DForOutWhenUnconnected=off
  wires:
  Switch/1 -> Gain4/1  "A"
  Add/1 -> Switch1/2
  Gain/1 -> Add1/1, Add/1
  Gain3/1 -> Add2/2
  Gain2/1 -> Add2/3
  Constant/1 -> Switch/1, Switch2/1, Switch1/1
  Add1/1 -> Switch2/2
  Gain1/1 -> Add1/2, Add/2
  Add2/1 -> MATLAB Function/1(u)
  Constant1/1 -> Switch2/3, Switch1/3, Switch/3
  Gain4/1 -> Add2/1
  beta/1 -> Switch/2, Gain1/1
  Switch2/1 -> Gain2/1  "C"
  Switch1/1 -> Gain3/1  "B"
  alpha/1 -> Gain/1
  MATLAB Function/1(y) -> N/1

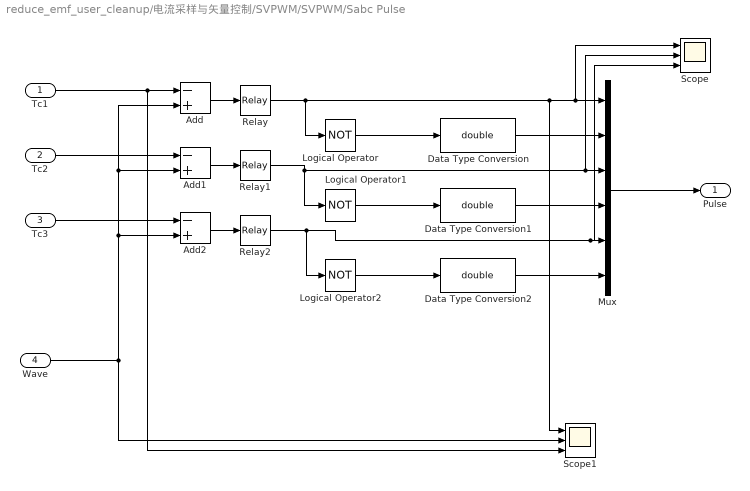
== system reduce_emf_user_cleanup/电流采样与矢量控制/SVPWM/SVPWM/Sabc Pulse ==
  Tc1 : Inport
  Tc2 : Inport  Port=2
  Tc3 : Inport  Port=3
  Wave : Inport  Port=4
  Add : Sum  Inputs=-+
  Add1 : Sum  Inputs=-+
  Add2 : Sum  Inputs=-+
  Data Type Conversion : DataTypeConversion  OutDataTypeStr=double  SaturateOnIntegerOverflow=off  RndMeth=Floor
  Data Type Conversion1 : DataTypeConversion  OutDataTypeStr=double  SaturateOnIntegerOverflow=off  RndMeth=Floor
  Data Type Conversion2 : DataTypeConversion  OutDataTypeStr=double  SaturateOnIntegerOverflow=off  RndMeth=Floor
  Logical Operator : Logic  Operator=NOT  AllPortsSameDT=off  OutDataTypeStr=boolean
  Logical Operator1 : Logic  Operator=NOT  AllPortsSameDT=off  OutDataTypeStr=boolean
  Logical Operator2 : Logic  Operator=NOT  AllPortsSameDT=off  OutDataTypeStr=boolean
  Mux : Mux  Inputs=6
  Relay : Relay
  Relay1 : Relay
  Relay2 : Relay
  Scope : Scope  NumInputPorts=3
  Scope1 : Scope  NumInputPorts=3
  "Pulse " : Outport  VectorParamsAs1DForOutWhenUnconnected=off
  wires:
  Add/1 -> Relay/1
  Add1/1 -> Relay1/1
  Wave/1 -> Add2/2, Add1/2, Add/2, Scope1/2
  Tc2/1 -> Add1/1
  Tc1/1 -> Scope1/3, Add/1
  Tc3/1 -> Add2/1
  Logical Operator/1 -> Data Type Conversion/1
  Logical Operator1/1 -> Data Type Conversion1/1
  Add2/1 -> Relay2/1
  Logical Operator2/1 -> Data Type Conversion2/1
  Mux/1 -> "Pulse "/1
  Relay/1 -> Scope1/1, Scope/1, Mux/1, Logical Operator/1
  Relay1/1 -> Scope/2, Mux/3, Logical Operator1/1
  Relay2/1 -> Logical Operator2/1, Scope/3, Mux/5
  Data Type Conversion/1 -> Mux/2
  Data Type Conversion1/1 -> Mux/4
  Data Type Conversion2/1 -> Mux/6

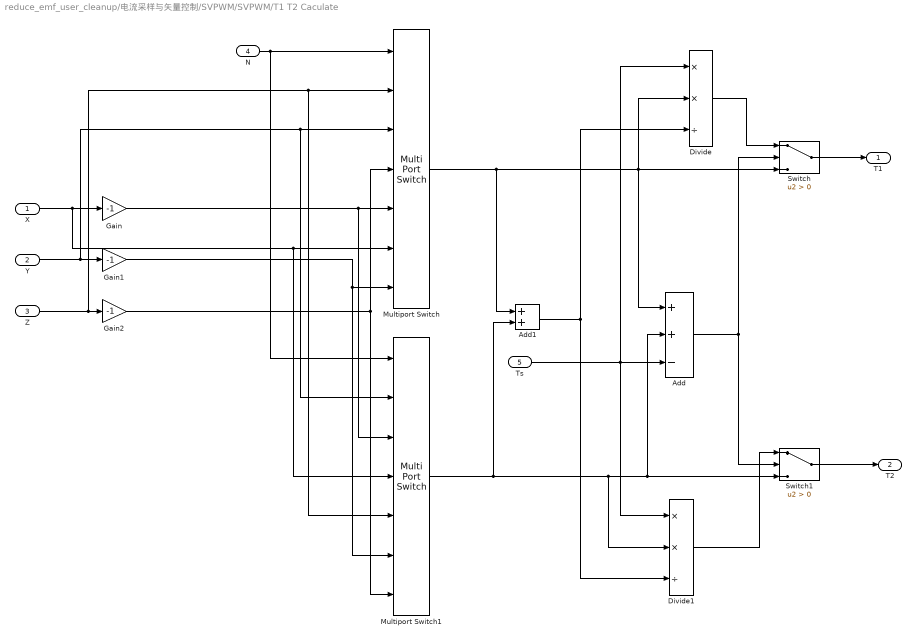
== system reduce_emf_user_cleanup/电流采样与矢量控制/SVPWM/SVPWM/T1 T2 Caculate ==
  X : Inport
  Y : Inport  Port=2
  Z : Inport  Port=3
  N : Inport  Port=4
  "Ts " : Inport  Port=5
  Add : Sum  Inputs=++-
  Add1 : Sum
  Divide : Product  Inputs=**/
  Divide1 : Product  Inputs=**/
  Gain : Gain  Gain=-1
  Gain1 : Gain  Gain=-1
  Gain2 : Gain  Gain=-1
  Multiport Switch : MultiPortSwitch  Inputs=6  SaturateOnIntegerOverflow=off  InputSameDT=off
  Multiport Switch1 : MultiPortSwitch  Inputs=6  SaturateOnIntegerOverflow=off  InputSameDT=off
  Switch : Switch  Criteria=u2 > Threshold  SaturateOnIntegerOverflow=off  InputSameDT=off
  Switch1 : Switch  Criteria=u2 > Threshold  SaturateOnIntegerOverflow=off  InputSameDT=off
  T1 : Outport  VectorParamsAs1DForOutWhenUnconnected=off
  T2 : Outport  Port=2  VectorParamsAs1DForOutWhenUnconnected=off
  wires:
  Y/1 -> Multiport Switch1/2, Multiport Switch/3, Gain1/1
  X/1 -> Multiport Switch1/4, Multiport Switch/6, Gain/1
  N/1 -> Multiport Switch/1, Multiport Switch1/1
  Z/1 -> Multiport Switch1/5, Multiport Switch/2, Gain2/1
  Gain2/1 -> Multiport Switch1/7, Multiport Switch/4
  Gain/1 -> Multiport Switch1/3, Multiport Switch/5
  Gain1/1 -> Multiport Switch1/6, Multiport Switch/7
  Multiport Switch/1 -> Add1/1, Divide/2, Add/1, Switch/3
  Multiport Switch1/1 -> Add1/2, Divide1/2, Add/2, Switch1/3
  "Ts "/1 -> Divide1/1, Divide/1, Add/3
  Add/1 -> Switch1/2, Switch/2
  Divide/1 -> Switch/1
  Add1/1 -> Divide/3, Divide1/3
  Switch/1 -> T1/1
  Switch1/1 -> T2/1
  Divide1/1 -> Switch1/1

== system reduce_emf_user_cleanup/电流采样与矢量控制/SVPWM/SVPWM/Tc Caculate ==
  T1 : Inport
  T2 : Inport  Port=2
  Ts : Inport  Port=3
  N : Inport  Port=4
  Multiport Switch : MultiPortSwitch  Inputs=6  SaturateOnIntegerOverflow=off  InputSameDT=off
  Multiport Switch1 : MultiPortSwitch  Inputs=6  SaturateOnIntegerOverflow=off  InputSameDT=off
  Multiport Switch2 : MultiPortSwitch  Inputs=6  SaturateOnIntegerOverflow=off  InputSameDT=off
  Mux : Mux  Inputs=3
  Scope : Scope  NumInputPorts=3
  Ta : Fcn  Expr=(u(3)-u(1)-u(2))/4
  Tb : Fcn  Expr=(u(3)-u(2)+u(1))/4
  Tc : Fcn  Expr=(u(3)+u(2)+u(1))/4
  Tc1 : Outport  VectorParamsAs1DForOutWhenUnconnected=off
  Tc2 : Outport  Port=2  VectorParamsAs1DForOutWhenUnconnected=off
  Tc3 : Outport  Port=3  VectorParamsAs1DForOutWhenUnconnected=off
  wires:
  T2/1 -> Mux/2
  T1/1 -> Mux/1
  Ts/1 -> Mux/3
  Mux/1 -> Tc/1, Ta/1, Tb/1
  N/1 -> Multiport Switch2/1, Multiport Switch1/1, Multiport Switch/1
  Ta/1 -> Multiport Switch2/7, Multiport Switch2/5, Multiport Switch/3, Multiport Switch/4, Multiport Switch1/6, Multiport Switch1/2
  Tb/1 -> Multiport Switch/7, Multiport Switch/2, Multiport Switch1/4, Multiport Switch2/6, Multiport Switch2/3, Multiport Switch1/5
  Tc/1 -> Multiport Switch2/4, Multiport Switch2/2, Multiport Switch1/7, Multiport Switch1/3, Multiport Switch/6, Multiport Switch/5
  Multiport Switch/1 -> Scope/1, Tc1/1
  Multiport Switch1/1 -> Scope/2, Tc2/1
  Multiport Switch2/1 -> Scope/3, Tc3/1

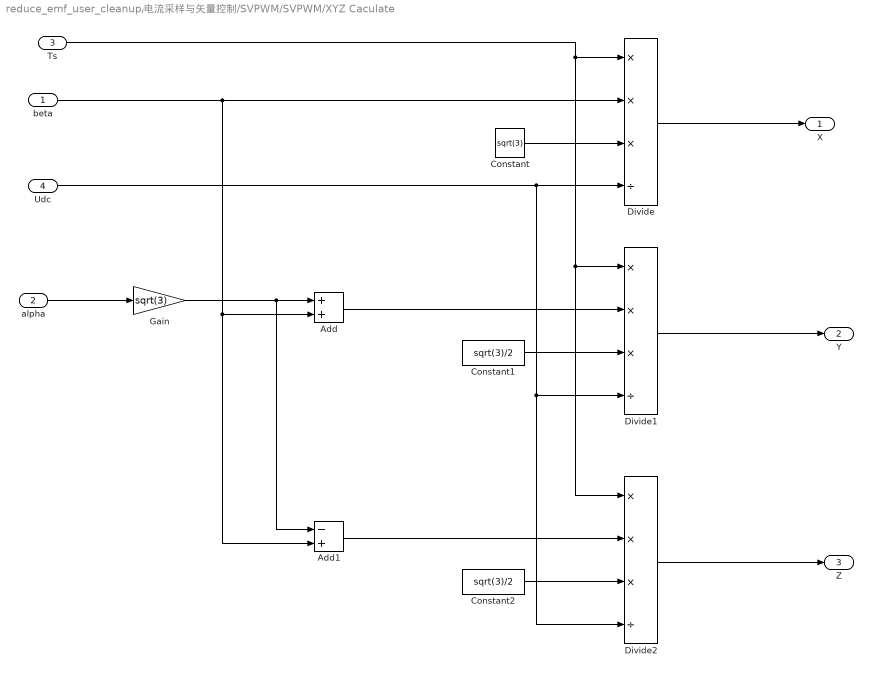
== system reduce_emf_user_cleanup/电流采样与矢量控制/SVPWM/SVPWM/XYZ Caculate ==
  beta : Inport
  alpha : Inport  Port=2
  "Ts " : Inport  Port=3
  Udc : Inport  Port=4
  Add : Sum
  Add1 : Sum  Inputs=-+
  Constant : Constant  Value=sqrt(3)
  Constant1 : Constant  Value=sqrt(3)/2
  Constant2 : Constant  Value=sqrt(3)/2
  Divide : Product  Inputs=***/
  Divide1 : Product  Inputs=***/
  Divide2 : Product  Inputs=***/
  Gain : Gain  Gain=sqrt(3)
  X : Outport  VectorParamsAs1DForOutWhenUnconnected=off
  Y : Outport  Port=2  VectorParamsAs1DForOutWhenUnconnected=off
  Z : Outport  Port=3  VectorParamsAs1DForOutWhenUnconnected=off
  wires:
  "Ts "/1 -> Divide2/1, Divide1/1, Divide/1
  Udc/1 -> Divide1/4, Divide2/4, Divide/4
  Constant/1 -> Divide/3
  beta/1 -> Add1/2, Add/2, Divide/2
  Constant2/1 -> Divide2/3
  Constant1/1 -> Divide1/3
  Add/1 -> Divide1/2
  Add1/1 -> Divide2/2
  Gain/1 -> Add1/1, Add/1
  alpha/1 -> Gain/1
  Divide1/1 -> Y/1
  Divide/1 -> X/1
  Divide2/1 -> Z/1

== matlab function reduce_emf_user_cleanup/电流采样与矢量控制/SVPWM/SVPWM/N Caculate/MATLAB Function ==
  data: u input; y output
function y = fcn(u)
if u==0
    y=1;
else
    y = u;
end

== matlab function reduce_emf_user_cleanup/MATLAB Function2 ==
  data: n input; n_filt output
function n_filt = fcn(n)
%#codegen
% 五路共用相同的50 Hz低通；周期平均在参数辨识函数内部执行。
n_filt=n;
end

== matlab function reduce_emf_user_cleanup/反电动势观测与锁相环/MATLAB Function1 ==
  data: n input; n_filt output
function n_filt = fcn(n)
%#codegen
% 文档图12.2的PLL速度反馈接口；输入来自原有一拍延迟的PLL速度。
% 本版旁路原100Hz低通，确保角度推进与解耦使用同一拍速度。
n_filt = n;
end

== matlab function reduce_emf_user_cleanup/备用模型_已停用/Subsystem/MATLAB Function1 ==
  data: u input; y output; deta input
function y = fcn(u,deta)
a=1e-6;
if u<a
    y=0;
else
    y=deta;
end

== matlab function reduce_emf_user_cleanup/反电动势观测与锁相环/锁相环1/MATLAB Function ==
  settings: updateMethod=DISCRETE  sampleTime=1e-4
  data: Ed_hat input size=1; Eq_hat input size=1; theta output size=1; we output size=1; IF_sensorless_mode input; id_offset output; vfl_state output; sample_ack input
function [theta, we, id_offset, vfl_state] = fcn(Ed_hat, Eq_hat, ...
                                                  IF_sensorless_mode, sample_ack)
%#codegen
% 无位置传感器 PLL + 参数辨识注入状态机
%   1) 用反电动势 Ed/Eq 估计电角度 theta、电角速度 we（式 12.7 的 PLL）
%   2) 切到无感后，按固定时长分 6 段注入 ±虚拟反电动势并改工作点，
%      配合外部采样做参数辨识
%--------------------------------------------------------------------------

% ---- 控制与 PLL 常数 ----
Ts      = 1e-4;      % 控制周期 100 us
wn      = 50;        % PLL 带宽, rad/s
zeta    = 0.707;     % 阻尼比
kp      = 2*zeta*wn; % PI 比例增益
ki      = wn*wn;     % PI 积分增益
we_max  = 1256;      % 电角速度限幅, rad/s
E_min   = 1e-3;      % 反电动势太小则不更新相位误差, V
EQ_EPS  = 1e-6;      % Eq 分母防除零

% ---- 状态机时序（单位：控制周期数）----
T_SETTLE  = 5000;    % I/F→无感 建立时间 0.5 s
T_SEG     = 6000;    % 普通采样段    0.6 s
T_WORKPT  = 10000;   % 工作点段      1.0 s
CAL_START = 1500;    % 标定脉冲起点 0.15 s
CAL_STOP  = 3500;    % 标定脉冲终点 0.35 s
CAL_AMP   = 0.2;     % 标定脉冲幅值, A
CAL_LEN   = 0.2;     % 标定脉冲时长, s
ID_TARGET = -1.0;    % 工作点 d 轴偏移, A
ID_SLEW   = 10;      % id 斜坡速率, A/s

% ---- 状态编号 ----
S_IDLE   = 0;    % 等待无感建立
S_BASE   = 2;    % 基线/准备段
S_INJ_P  = 3;    % +amp 注入
S_INJ_N  = 4;    % -amp 注入
S_WORKPT = 5;    % 切工作点（含标定脉冲）
S_RECOV  = 6;    % 恢复段
S_WKP_P  = 7;    % 新工作点 +amp
S_WKP_N  = 8;    % 新工作点 -amp
S_DONE   = 9;    % 结束
S_ABORT  = 10;   % 数值错误中止

% ---- 持久状态 ----
persistent theta_z speed_i state tick stable amp id_ramp
if isempty(theta_z)
    theta_z = 0;  speed_i = 0;  state = S_IDLE;
    tick = 0;     stable  = 0;  amp = 0;   id_ramp = 0;
end

% ---- 输入保护 ----
if ~isfinite(Ed_hat) || ~isfinite(Eq_hat) || ~isfinite(IF_sensorless_mode)
    Ed_hat = 0;  Eq_hat = 0;  IF_sensorless_mode = 0;
end

% ================= 状态机 =================
injection = 0;        % 注入到 PLL 的 Ed 的虚拟反电动势
id_target = 0;        % id 斜坡目标值

if IF_sensorless_mode < 0.5 || ~isfinite(Ed_hat + Eq_hat)
    % 退出无感或输入异常：复位
    state = S_IDLE;  tick = 0;  stable = 0;
end

if state > 0
    tick = tick + 1;

    if state >= S_BASE && state <= S_WKP_N && sample_ack < 0
        % 外部报数值错误：中止
        state = S_ABORT;  tick = 0;

    elseif state == S_WORKPT && tick > T_WORKPT
        % 工作点段较慢，单独用 1 s
        state = S_RECOV;  tick = 1;
        amp = min(0.6, max(0.2, 0.01*abs(Eq_hat)));

    elseif state >= S_BASE && state <= S_WKP_N && state ~= S_WORKPT && tick > T_SEG
        % 普通段 0.6 s 后前进
        state = state + 1;  tick = 1;
    end

    % 5~8 段施加 d 轴工作点偏移
    if state >= S_WORKPT && state <= S_WKP_N
        id_target = ID_TARGET;
    end

    % 3/7 正向注入， 4/8 反向注入
    if state == S_INJ_P || state == S_WKP_P
        injection = amp;
    elseif state == S_INJ_N || state == S_WKP_N
        injection = -amp;
    end
end

% ---- id 斜坡（10 A/s）----
if IF_sensorless_mode < 0.5 || state == S_ABORT
    id_ramp = 0;
else
    id_step = ID_SLEW * Ts;
    id_ramp = id_ramp + min(max(id_target - id_ramp, -id_step), id_step);
end

% ---- 工作点段内的 200 mA 标定脉冲（分离 R 与逆变器压降）----
id_calibration = 0;
if state == S_WORKPT && tick >= CAL_START && tick <= CAL_STOP
    t_pulse = (tick - CAL_START) * Ts;
    envelope = sin(pi*t_pulse/CAL_LEN)^2;
    id_calibration = CAL_AMP * envelope * cos(theta_z);
end

id_offset = id_ramp + id_calibration;
vfl_state = int32(state);

% ================= PLL =================
Ed_pll = Ed_hat + injection;     % 注入只影响 PLL，不改变电机电压命令

if Ed_hat*Ed_hat + Eq_hat*Eq_hat > E_min*E_min
    % 式(12.7)：phase_error = atan(-Ed/Eq)，Eq 做数值正则化
    eq_safe = Eq_hat;
    if abs(eq_safe) < EQ_EPS
        eq_safe = sign(eq_safe + (eq_safe == 0)) * EQ_EPS;  % 0 时取 +EPS
    end
    phase_error = atan(-Ed_pll / eq_safe);
else
    phase_error = 0;
end

% PI → 电角速度（带条件积分抗饱和）
we_unsat = speed_i + kp*phase_error;
we = min(max(we_unsat, -we_max), we_max);

if (we_unsat <= we_max && we_unsat >= -we_max) || ...
   (we_unsat >  we_max && phase_error < 0)     || ...
   (we_unsat < -we_max && phase_error > 0)
    speed_i = speed_i + ki*Ts*phase_error;
end
speed_i = min(max(speed_i, -we_max), we_max);

% ---- 角度积分（输出滞后一拍，避免代数环）----
theta   = theta_z;
theta_z = mod(theta_z + Ts*we, 2*pi);

% ================= I/F → 无感 =================
if state == S_IDLE && IF_sensorless_mode >= 0.5
    stable = stable + 1;
    if stable >= T_SETTLE
        state = S_BASE;  tick = 0;  stable = 0;
        amp = min(0.6, max(0.2, 0.01*abs(Eq_hat)));
    end
elseif state == S_IDLE
    stable = 0;
end
end

== matlab function reduce_emf_user_cleanup/反电动势观测与锁相环/反电动势观测器 ==
  data: ua input; Ed_hat output; ub input; ia input; ib input; Eq_hat output; we input; theta_hat output; we_out output; theta_z1 input
function [Ed_hat,Eq_hat,theta_hat,we_out] = fcn_improved_paper_strict(ua,ub,ia,ib,we,theta_z1)
%#codegen
%==================================================
% 文档式(12.5)、(12.6)及图12.2：dq降阶扩展反电动势观测器。
% 当前对象为SPMSM，Ld=Lq=Ls，扩展反电动势即永磁体反电动势。
% 输入ua/ub、ia/ib为alpha-beta电压和电流，we为延迟一拍的PLL电角速度。
% theta_z1为延迟一拍的PLL角度，先按同一拍we推进至当前时刻。
% 输出Ed_hat/Eq_hat单位V，直接送入反电动势PLL，不再转换成磁链。
%==================================================
persistent zd zq bd_old bq_old
Ts = 1e-4;                    % 原模型控制周期，s
Ls = 8.96e-3;                 % 参考电感，H
Rs = 1.8665;                  % 参考电阻，ohm
Gr = 500;                     % 所选观测器增益初值，rad/s；文档未给定数值

% 将延迟角度推进一拍，与本周期电压、电流对齐。
theta_c = mod(theta_z1+Ts*we,2*pi);
cs = cos(theta_c);
sn = sin(theta_c);
ud =  cs*ua+sn*ub;
uq = -sn*ua+cs*ub;
id =  cs*ia+sn*ib;
iq = -sn*ia+cs*ib;

% 文档式(12.6)的解耦电压。
ud1 = ud+we*Ls*iq;
uq1 = uq-we*Ls*id;

% 图12.2的降阶实现：
% E_hat = Gr/(s+Gr) * (u_dq1-Rs*i_dq-Ls*p*i_dq)。
% 定义z=E_hat+Gr*Ls*i，消除显式电流微分：
% z_dot=-Gr*z+Gr*(u_dq1+(Gr*Ls-Rs)*i_dq)。
% 两个轴独立，采用梯形法离散，保持100us控制周期。
bd = Gr*(ud1+(Gr*Ls-Rs)*id);
bq = Gr*(uq1+(Gr*Ls-Rs)*iq);
if isempty(zd)
    zd = Gr*Ls*id;            % 初始Ed_hat=0
    zq = Gr*Ls*iq;            % 初始Eq_hat=0
    bd_old = bd;
    bq_old = bq;
else
    a = 0.5*Ts*Gr;
    zd = ((1-a)*zd+0.5*Ts*(bd+bd_old))/(1+a);
    zq = ((1-a)*zq+0.5*Ts*(bq+bq_old))/(1+a);
    bd_old = bd;
    bq_old = bq;
end
Ed_hat = zd-Gr*Ls*id;
Eq_hat = zq-Gr*Ls*iq;

% 辅助监测输出，主闭环只使用前两路反电动势。
if abs(Ed_hat)+abs(Eq_hat)>1e-6
    eq_safe = Eq_hat;
    if abs(eq_safe)<1e-6
        if eq_safe>=0
            eq_safe=1e-6;
        else
            eq_safe=-1e-6;
        end
    end
    theta_hat = mod(theta_c+atan(-Ed_hat/eq_safe),2*pi);
else
    theta_hat = theta_c;
end
we_out = we;
end
